simulink model "temp"  (Simulink 7.7)
settings: Solver=FixedStepDiscrete  SolverMode=SingleTasking  StartTime=0.0  StopTime=10.0  FixedStep=0.001  RelTol=1e-3
libraries: dsPICdrivers x8, simulink x1, simulink_need_slupdate x1
settings Model: Creator=Bryant  LastModifiedBy=Lubin
settings OptimizationCC: OptimizeModelRefInitCode=on  LifeSpan=1
settings HardwareCC: ProdBitPerInt=16  ProdBitPerPointer=16  ProdEndianess=LittleEndian  ProdWordSize=16  ProdHWDeviceType=16-bit Generic
settings RTWCC: SystemTargetFile=dspic.tlc  MakeCommand=make_CreateMPLAB  TemplateMakefile=dspic_pic30_gcc.tmf  PostCodeGenCommand=dsPIC_Compile()  Description=Embedded Target for Microchip dsPIC (real-time)  ProcessScript=dspic_make_rtw_hook
settings CodeAppCC: IgnoreCustomStorageClasses=off
settings STFCustomTargetCC: FunctionExecutionProfile=off  IncludeMdlTerminateFcn=off  CombineOutputUpdateFcns=on  SuppressErrorStatus=on  ERTCustomFileBanners=on  SupportContinuousTime=off  SupportNonInlinedSFcns=off  SystemTargetFile=dspic.tlc
settings ERTTargetCC: FunctionExecutionProfile=off  MultiwordLength=2048  ParMdlRefBuildCompliant=off  CompOptLevelCompliant=off  IncludeMdlTerminateFcn=off  SuppressErrorStatus=on  ERTFirstTimeCompliant=off  ModelStepFunctionPrototypeControlCompliant=off  CPPClassGenCompliant=off  InlinedParameterPlacement=NonHierarchical  ERTSrcFileBannerTemplate=dsPIC_code_template.cgt  ERTHdrFileBannerTemplate=dsPIC_code_template.cgt  ERTDataSrcFileTemplate=dsPIC_code_template.cgt  ERTDataHdrFileTemplate=dsPIC_code_template.cgt  ERTCustomFileTemplate=dsPIC_main.tlc  ConvertIfToSwitch=off
settings CustomProperty: DataType=string  Value=C:\PROGRA~1\MATLAB\R2011a\bin\win64\gmake

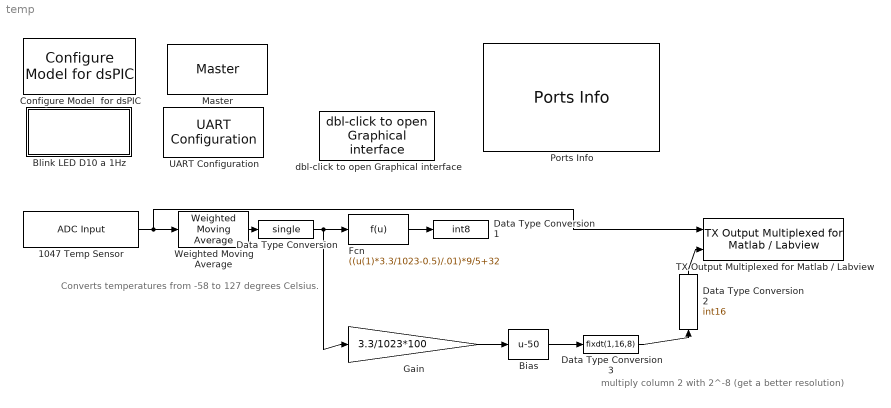
== system temp ==
  note: Converts temperatures from -58 to 127 degrees Celsius.
  note: multiply column 2 with 2^-8 (get a better resolution)
  1047 Temp Sensor : dsPICdrivers/Peripheral I//O/ADC Input  Tag=dsPIC_ADC  Priority=5  ADC_TYPE=10 bits  ADC_MODE=Continuous sampling & get last channel value  NbrSampleStep=1  VoltRefpopup="AVdd  -  AVss"  OutFormatBitspopup=0000 00dd dddd dddd : Integer  InterruptPriority=6  ANCHANNELS=[4]  MaxName=ANmax = 1023  Rin=1e2  ADCS=12  SAMC=1  Temperature=25  DMAChannel=7  SampleTime=.01  Status="OK  |  Tsmp=1.625e-007 |  T/Channel=2.113e-006 |  Tall=2.113e-006"  SSRC=auto convert
  Bias : Bias  Bias=-50
  Blink LED D10 a 1Hz : Subsystem
      mask Display: disp('blink');
  Configure Model  for dsPIC : dsPICdrivers/Simulink Configuration/Configure Model  for dsPIC
  Data Type Conversion : DataTypeConversion  OutDataTypeStr=single
  Data Type Conversion1 : DataTypeConversion  OutDataTypeStr=int8
  Data Type Conversion2 : DataTypeConversion  OutDataTypeStr=int16  ConvertRealWorld=Stored Integer (SI)
  Data Type Conversion3 : DataTypeConversion  OutDataTypeStr=fixdt(1,16,8)
  Fcn : Fcn  Expr=((u(1)*3.3/1023-0.5)/.01)*9/5+32
  Gain : Gain  Gain=3.3/1023*100
  Master : dsPICdrivers/Master  Tag=dsPIC_MASTER  Priority=1  TimeStepType=Timer1  picType=33fJ256GP710  fcy=40000000  Quartz_33f=8e6  PLLActive_33f=on  fcyDesired_33f=40000000  tmr1="[1  39999  0]"  tmr1Info="Time Step : 0.001  ;   Error : 0%  PR1=39999"  tmr2345="[0  0  0  0  0  0  0  0]"  tmr2345cfg=[-1 -1 -1 -1 -1 -1 -1 -1]  IOautoConf=on  typePort="[ 0   0   0   0   0   0   0  10   0   0   0   0   0   0   0   0   0   0   0   0   8   0   0   0   0   0   0   0   0   0   0   0   0   0   0   0   0   0   0   0   0   0   0   0   0   0   0   0   0   0   0   0   0   0   0   0   0   0   0   0   0   0   0   0   0   0   0   0   0   0   0   0   0   0   0   0   0   0   0   0   0   0   0   0   4   5   0   0   0   0   0   0   0   0   0   0   0   0   0   0   0   0   0   0   0   0   0   0   0   0   0   0 ]"  TRIS="[ 65407  65535  65535  65535  65535  65535  65535 ]"  ADPCFG=8388608  MasterBusyPort=None  MasterOverloadPort=None  FOSC=Quartz (XT - HS)  ClockSwitchMonitor=Both disabled  TempProtection_33f=TEMP_ON  FPBOR=<empty>  PWRT=disable  MCLR=<empty>  ICD=ICS_PGD1  JTAGEN=JTAGEN_OFF  PowerSave=off  OverrideFcy=off  NewFcy=1e6  PR2345="[65535  65535  65535  65535  65535  65535  65535  65535]"
  Ports Info : dsPICdrivers/Ports Info  Tag=dsPIC_PortInfo
  TX Output Multiplexed for Matlab / Labview : dsPICdrivers/Serial PORT/TX Output Multiplexed for Matlab // Labview  Tag=dsPIC_TX_Multiplexed  Priority=5  UART=2  CleverSpreadingChk=on  CleverSpreading=1  CHANNEL=[0 1]  CHANNELBLOCKED=[]  CHANNELBLOCKED_BITEWISE=0  Status=OK
  UART Configuration : dsPICdrivers/Serial PORT/UART Configuration  Tag=dsPIC_config_UART  Priority=2  UART=2  proposed_BAUD=115200  BAUD=115200  ALT_TX_RX=on  InterruptTxWhen=When Transmit Buffer is empty  TXInterruptPri=1  TxBufferSize=32  TXEN=on  InterruptRxWhen=When Receive Buffer is full (contain 4 characters)  RXInterruptPri=2  RxBufferSize=32  DoNotImplementRxInterrupt=off  DoNotImplementTxInterrupt=off  UxBRG=21  Info="UxBRG = 21   ||  Real Baud : 113636   ||  % error : -1.3573  ||  max 11.3636 Bytes / Step"  RealBaud=0  ERROR=-1.3573  BYTES_STEP=11.3636
  Weighted Moving Average : simulink_need_slupdate/Weighted Moving Average  mgainval=[.2 .2 .2 .2 .2]  vinit=0.0  samptime=-1  OutDataTypeStr=Inherit: Inherit via back propagation  OutDataType=sfix(16)  OutScaling=2^-10  DoSatur=off  GainDataType=uint(16)  MatRadixGroup=Best Precision: Matrix-wise  GainScaling=2^-10
  dbl-click to open Graphical interface : dsPICdrivers/Serial PORT/dbl-click to open Graphical interface  Nothing=0
  wires:
  1047 Temp Sensor/1 -> Weighted Moving Average/1, TX Output Multiplexed for Matlab / Labview/1
  Weighted Moving Average/1 -> Data Type Conversion/1
  Fcn/1 -> Data Type Conversion1/1
  Data Type Conversion/1 -> Fcn/1, Gain/1
  Gain/1 -> Bias/1
  Bias/1 -> Data Type Conversion3/1
  Data Type Conversion3/1 -> Data Type Conversion2/1
  Data Type Conversion2/1 -> TX Output Multiplexed for Matlab / Labview/2

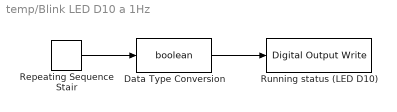
== system temp/Blink LED D10 a 1Hz ==
  Data Type Conversion : DataTypeConversion  OutDataTypeStr=boolean  RndMeth=Simplest
  Repeating Sequence Stair : simulink/Sources/Repeating Sequence Stair  SystemSampleTime=-1  OutValues=[1 0]  tsamp=1  OutMin=[]  OutMax=[]  OutDataTypeStr=double  OutputDataTypeScalingMode=double  OutDataType=fixdt(0,8)  ConRadixGroup=Best Precision: Vector-wise  OutScaling=2^-12
  Running status (LED D10) : dsPICdrivers/Digital I//O/Digital Output Write  Tag=dsPIC_Digital_Output  Priority=5  PORT=A  Pin=[7]  Simultaneous=off  OrderingInOutPopup=None
  wires:
  Repeating Sequence Stair/1 -> Data Type Conversion/1
  Data Type Conversion/1 -> Running status (LED D10)/1
